simulink model "P5NP"  (R2023b)
settings: Solver=VariableStepAuto  StartTime=0.0  StopTime=20  RelTol=1e-3
settings Model: Creator=joser  LastModifiedBy=joser
settings ModelReferenceCC: EnableRefExpFcnMdlSchedulingChecks=on

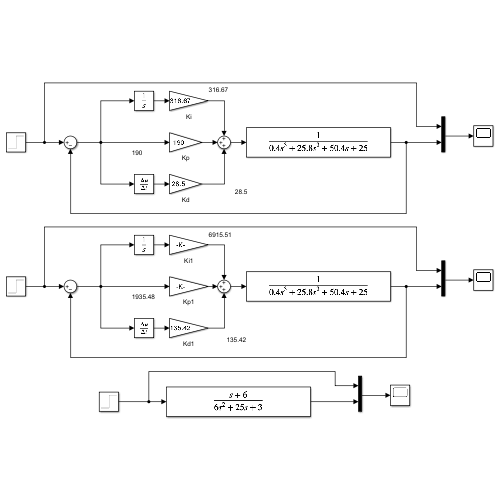
[thumbnail: Simulink's stored preview of the top-level diagram]
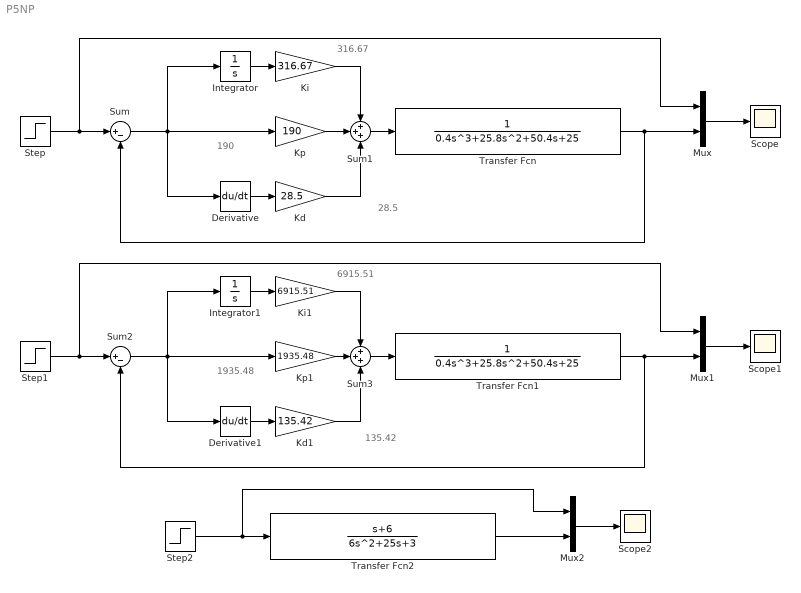
== system P5NP ==
  note: 316.67
  note: 190
  note: 28.5
  note: 6915.51
  note: 135.42
  note: 1935.48
  Derivative : Derivative
  Derivative1 : Derivative
  Integrator : Integrator
  Integrator1 : Integrator
  Kd : Gain  Gain=28.5
  Kd1 : Gain  Gain=135.42
  Ki : Gain  Gain=316.67
  Ki1 : Gain  Gain=6915.51
  Kp : Gain  Gain=190
  Kp1 : Gain  Gain=1935.48
  Mux : Mux  Inputs=2
  Mux1 : Mux  Inputs=2
  Mux2 : Mux  Inputs=2
  Scope : Scope
  Scope1 : Scope
  Scope2 : Scope
  Step : Step  SampleTime=0
  Step1 : Step  SampleTime=0
  Step2 : Step  SampleTime=0
  Sum : Sum  Inputs=|+-
  Sum1 : Sum  Inputs=+++
  Sum2 : Sum  Inputs=|+-
  Sum3 : Sum  Inputs=+++
  Transfer Fcn : TransferFcn  Denominator=[0.4 25.8 50.4 25]
  Transfer Fcn1 : TransferFcn  Denominator=[0.4 25.8 50.4 25]
  Transfer Fcn2 : TransferFcn  Numerator=[1 6]  Denominator=[6 25 3]
  wires:
  Step/1 -> Mux/1, Sum/1
  Transfer Fcn/1 -> Mux/2, Sum/2
  Sum1/1 -> Transfer Fcn/1
  Mux/1 -> Scope/1
  Sum/1 -> Derivative/1, Integrator/1, Kp/1
  Kp/1 -> Sum1/2
  Ki/1 -> Sum1/1
  Kd/1 -> Sum1/3
  Integrator/1 -> Ki/1
  Derivative/1 -> Kd/1
  Integrator1/1 -> Ki1/1
  Kp1/1 -> Sum3/2
  Sum2/1 -> Derivative1/1, Integrator1/1, Kp1/1
  Mux1/1 -> Scope1/1
  Kd1/1 -> Sum3/3
  Sum3/1 -> Transfer Fcn1/1
  Derivative1/1 -> Kd1/1
  Ki1/1 -> Sum3/1
  Step1/1 -> Mux1/1, Sum2/1
  Transfer Fcn1/1 -> Mux1/2, Sum2/2
  Transfer Fcn2/1 -> Mux2/2
  Mux2/1 -> Scope2/1
  Step2/1 -> Mux2/1, Transfer Fcn2/1
